simulink model "Geradeausfahrt"  (R2026b)
settings: Solver=FixedStepDiscrete  StopTime=inf  FixedStep=PAR_Sys_AbtastBasis_f64  EnableMultiTasking=on
StopFcn:
  | SpeichereGeradeausfahrt('Geradeausfahrt');
model workspace (MAT data in the model file):
  PAR_AktMot_PWM0_u8 = 80
  PAR_AktMot_RichtL_u8 = 0
  PAR_AktMot_RichtR_u8 = 1
  PAR_AktMot_Start_f32 = Simulink.Parameter
  PAR_AktMot_Start_f32.Value = 0
  PAR_AktMot_Start_f32.Complexity = 'real'
  PAR_AktMot_Start_f32.Dimensions = [1 1]
  PAR_AktMot_Start_f32.DataType = 'single'
  PAR_RegGer_Kp_f32 = Simulink.Parameter
  PAR_RegGer_Kp_f32.Value = 100
  PAR_RegGer_Kp_f32.Complexity = 'real'
  PAR_RegGer_Kp_f32.Dimensions = [1 1]
  PAR_RegGer_Kp_f32.DataType = 'single'
  PAR_RegGer_SSoll_f32 = 8
  PAR_SenOdo_IncU_f32 = 40
  PAR_SenOdo_KorrSL_f32 = 1
  PAR_SenOdo_RadR_f32 = 0.0320000015199
  PAR_SenOdo_Spur_f32 = 0.140000000596
  PAR_Sys_AbtastBasis_f64 = 0.01
  PAR_Sys_Abtast_f64 = 0.01
libraries: arduinolib x8
settings Model: SILPILModeSetting=veronly  SimulationMode=external
settings SolverCC: AutoInsertRateTranBlk=on
settings DataIOCC: ReturnWorkspaceOutputs=off
settings OptimizationCC: DifferentSizesBufferReuse=on  EfficientTunableParamExpr=on  EnhancedBackFolding=on  MaxStackSize=64  OptimizationCustomize=off  OptimizeBlockOrder=speed  PassReuseOutputArgsAs=Individual arguments  RemoveInternalMemoryZeroInit=on  RemoveRootLevelIOMemoryZeroInit=on
settings DebuggingCC: ParameterTunabilityLossMsg=error
settings HardwareCC: ProdHWDeviceType=ARM Compatible->ARM Cortex  ProdLargestAtomicFloat=Double  ProdLargestAtomicInteger=Long
settings SFSimCC: MATLABDynamicMemAlloc=off
settings RTWCC: BuildConfiguration=Faster Runs  Description=Embedded Coder  HardwareBoard=Arduino Uno R4 WiFi  SystemTargetFile=ert.tlc  TLCOptions=-aInlineSetEventsForThisBaseRateFcn=TLC_FALSE -aSuppressMultiTaskScheduler=TLC_FALSE -aRateBasedStepFcn=1  TemplateMakefile=ert_default_tmf  Toolchain=Arduino ARM M4
settings CodeAppCC: ForceParamTrailComments=on  IgnoreCustomStorageClasses=off  InsertBlockDesc=on  OperatorAnnotations=on  SFDataObjDesc=on  SimulinkDataObjDesc=on
settings ERTTargetCC: CombineSignalStateStructs=on  ExtModeAutomaticAllocSize=off  ExtModeIntrfLevel=Level2 - Open  ExtModeMexFile=ext_xcp  ExtModeStaticAlloc=on  SupportContinuousTime=on  SupportVariableSizeSignals=on

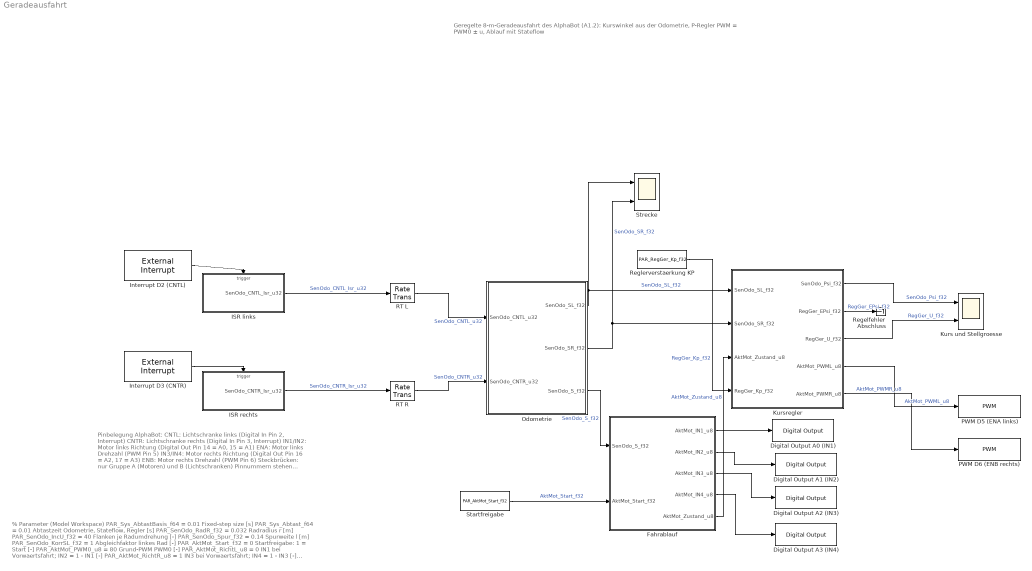
== system Geradeausfahrt ==
  note: % Parameter (Model Workspace)
      | PAR_Sys_AbtastBasis_f64 = 0.01 Fixed-step size [s]
      | PAR_Sys_Abtast_f64 = 0.01 Abtastzeit Odometrie, Stateflow, Regler [s]
      | PAR_SenOdo_RadR_f32 = 0.032 Radradius r [m]
      | PAR_SenOdo_IncU_f32 = 40 Flanken je Radumdrehung [-]
      | PAR_SenOdo_Spur_f32 = 0.14 Spurweite l [m]
      | PAR_SenOdo_KorrSL_f32 = 1 Abgleichfaktor linkes Rad [-]
      | PAR_AktMot_Start_f32 = 0 Startfreigabe: 1 = Start [-]
      | PAR_AktMot_PWM0_u8 = 80 Grund-PWM PWM0 [-]
      | PAR_AktMot_RichtL_u8 = 0 IN1 bei Vorwaertsfahrt; IN2 = 1 - IN1 [-]
      | PAR_AktMot_RichtR_u8 = 1 IN3 bei Vorwaertsfahrt; IN4 = 1 - IN3 [-]
      | PAR_RegGer_SSoll_f32 = 8 Sollstrecke [m]
      | PAR_RegGer_Kp_f32 = 100 Reglerverstae rkung KP [PWM/rad]
      |
      | % BSE_3: psi_k = psi_k-1 + (dsR - dsL) / l, e = 0 - psi, u = KP * e
      | PWML = PWM0 - u, PWMR = PWM0 + u
  note: Geregelte 8-m-Geradeausfahrt des AlphaBot (A1.2): Kurswinkel aus der Odometrie, P-Regler PWM = PWM0 ± u, Ablauf mit Stateflow
  note: Pinbelegung AlphaBot:
      | CNTL: Lichtschranke links (Digital In Pin 2, Interrupt)
      | CNTR: Lichtschranke rechts (Digital In Pin 3, Interrupt)
      | IN1/IN2: Motor links Richtung (Digital Out Pin 14 = A0, 15 = A1)
      | ENA: Motor links Drehzahl (PWM Pin 5)
      | IN3/IN4: Motor rechts Richtung (Digital Out Pin 16 = A2, 17 = A3)
      | ENB: Motor rechts Drehzahl (PWM Pin 6)
      | Steckbrücken: nur Gruppe A (Motoren) und B (Lichtschranken)
      | Pinnummern stehen direkt in den Blöcken (keine PAR_-Parameter).
  Digital Output A0 (IN1) : arduinolib/Digital Output  pinNumber=14  Direction=output  blockPlatform=arduino
  Digital Output A1 (IN2) : arduinolib/Digital Output  pinNumber=15  Direction=output  blockPlatform=arduino
  Digital Output A2 (IN3) : arduinolib/Digital Output  pinNumber=16  Direction=output  blockPlatform=arduino
  Digital Output A3 (IN4) : arduinolib/Digital Output  pinNumber=17  Direction=output  blockPlatform=arduino
  Fahrablauf : Stateflow chart  TreatAsAtomicUnit=on
  ISR links : Subsystem  TreatAsAtomicUnit=on
  ISR rechts : Subsystem  TreatAsAtomicUnit=on
  Interrupt D2 (CNTL) : arduinolib/External Interrupt  Pin=2  PullUp=off  Mode=CHANGE  InterruptSimulationInput=off
  Interrupt D3 (CNTR) : arduinolib/External Interrupt  Pin=3  PullUp=off  Mode=CHANGE  InterruptSimulationInput=off
  Kurs und Stellgroesse : Scope  NumInputPorts=2
      settings: ActiveDisplayYMinimum=-1.0587400176678445  ActiveDisplayYMaximum=1.3722724823321559
  Kursregler : MATLAB Function  TreatAsAtomicUnit=on
  Odometrie : MATLAB Function  TreatAsAtomicUnit=on
  PWM D5 (ENA links) : arduinolib/PWM  pinNumber=5  frequencyType=Default  desiredFrequency=490.2  achievableFrequency=490.2
  PWM D6 (ENB rechts) : arduinolib/PWM  pinNumber=6  frequencyType=Default  desiredFrequency=490.2  achievableFrequency=490.2
  RT L : RateTransition  Deterministic=off  OutPortSampleTime=PAR_Sys_Abtast_f64
  RT R : RateTransition  Deterministic=off  OutPortSampleTime=PAR_Sys_Abtast_f64
  Regelfehler Abschluss : Terminator
  Reglerverstaerkung KP : Constant  Value=PAR_RegGer_Kp_f32  OutDataTypeStr=single  SampleTime=PAR_Sys_Abtast_f64
  Startfreigabe : Constant  Value=PAR_AktMot_Start_f32  OutDataTypeStr=single  SampleTime=PAR_Sys_Abtast_f64
  Strecke : Scope  NumInputPorts=2
      settings: ActiveDisplayYMinimum=-0.329834002092661  ActiveDisplayYMaximum=1.9353644368944749
  wires:
  Interrupt D2 (CNTL)/1 -> ISR links/Trigger
  ISR links/1(SenOdo_CNTL_Isr_u32) -> RT L/1  "SenOdo_CNTL_Isr_u32"
  Interrupt D3 (CNTR)/1 -> ISR rechts/Trigger
  ISR rechts/1(SenOdo_CNTR_Isr_u32) -> RT R/1  "SenOdo_CNTR_Isr_u32"
  RT L/1 -> Odometrie/1(SenOdo_CNTL_u32)  "SenOdo_CNTL_u32"
  RT R/1 -> Odometrie/2(SenOdo_CNTR_u32)  "SenOdo_CNTR_u32"
  Odometrie/3(SenOdo_S_f32) -> Fahrablauf/1(SenOdo_S_f32)  "SenOdo_S_f32"
  Startfreigabe/1 -> Fahrablauf/2(AktMot_Start_f32)  "AktMot_Start_f32"
  Odometrie/1(SenOdo_SL_f32) -> Kursregler/1(SenOdo_SL_f32), Strecke/1  "SenOdo_SL_f32"
  Odometrie/2(SenOdo_SR_f32) -> Kursregler/2(SenOdo_SR_f32), Strecke/2  "SenOdo_SR_f32"
  Fahrablauf/5(AktMot_Zustand_u8) -> Kursregler/3(AktMot_Zustand_u8)  "AktMot_Zustand_u8"
  Reglerverstaerkung KP/1 -> Kursregler/4(RegGer_Kp_f32)  "RegGer_Kp_f32"
  Kursregler/4(AktMot_PWML_u8) -> PWM D5 (ENA links)/1  "AktMot_PWML_u8"
  Kursregler/5(AktMot_PWMR_u8) -> PWM D6 (ENB rechts)/1  "AktMot_PWMR_u8"
  Fahrablauf/1(AktMot_IN1_u8) -> Digital Output A0 (IN1)/1
  Fahrablauf/2(AktMot_IN2_u8) -> Digital Output A1 (IN2)/1
  Fahrablauf/3(AktMot_IN3_u8) -> Digital Output A2 (IN3)/1
  Fahrablauf/4(AktMot_IN4_u8) -> Digital Output A3 (IN4)/1
  Kursregler/1(SenOdo_Psi_f32) -> Kurs und Stellgroesse/1  "SenOdo_Psi_f32"
  Kursregler/3(RegGer_U_f32) -> Kurs und Stellgroesse/2  "RegGer_U_f32"
  Kursregler/2(RegGer_EPsi_f32) -> Regelfehler Abschluss/1  "RegGer_EPsi_f32"

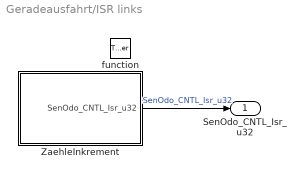
== system Geradeausfahrt/ISR links ==
  function : TriggerPort  TriggerType=function-call  VariantControl=(inherit)
  ZaehleInkrement : MATLAB Function  TreatAsAtomicUnit=on
  SenOdo_CNTL_Isr_u32 : Outport
  wires:
  ZaehleInkrement/1(SenOdo_CNTL_Isr_u32) -> SenOdo_CNTL_Isr_u32/1  "SenOdo_CNTL_Isr_u32"

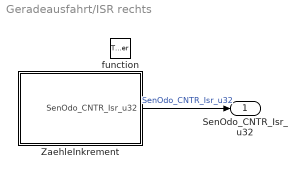
== system Geradeausfahrt/ISR rechts ==
  function : TriggerPort  TriggerType=function-call  VariantControl=(inherit)
  ZaehleInkrement : MATLAB Function  TreatAsAtomicUnit=on
  SenOdo_CNTR_Isr_u32 : Outport
  wires:
  ZaehleInkrement/1(SenOdo_CNTR_Isr_u32) -> SenOdo_CNTR_Isr_u32/1  "SenOdo_CNTR_Isr_u32"

== matlab function Geradeausfahrt/ISR rechts/ZaehleInkrement ==
  data: SenOdo_CNTR_Isr_u32 output
function SenOdo_CNTR_Isr_u32 = ZaehleInkrement()
% ZaehleInkrement: ISR je Flanke der Lichtschranke (Modus CHANGE)
% Ausgabe:  SenOdo_CNTR_Isr_u32 [1x1]: Flanken seit Programmstart [-]
persistent nZaehler   % Flankenzaehler [-]

if isempty(nZaehler)
    nZaehler = uint32(0);
end
nZaehler = nZaehler + 1;
SenOdo_CNTR_Isr_u32 = nZaehler;
end

== matlab function Geradeausfahrt/ISR links/ZaehleInkrement ==
  data: SenOdo_CNTL_Isr_u32 output
function SenOdo_CNTL_Isr_u32 = ZaehleInkrement()
% ZaehleInkrement: ISR je Flanke der Lichtschranke (Modus CHANGE)
% Ausgabe:  SenOdo_CNTL_Isr_u32 [1x1]: Flanken seit Programmstart [-]
persistent nZaehler   % Flankenzaehler [-]

if isempty(nZaehler)
    nZaehler = uint32(0);
end
nZaehler = nZaehler + 1;
SenOdo_CNTL_Isr_u32 = nZaehler;
end

== matlab function Geradeausfahrt/Odometrie ==
  settings: updateMethod=DISCRETE  sampleTime=PAR_Sys_Abtast_f64
  data: SenOdo_CNTL_u32 input; SenOdo_SL_f32 output; SenOdo_CNTR_u32 input; SenOdo_SR_f32 output; SenOdo_S_f32 output; PAR_SenOdo_RadR_f32 parameter; PAR_SenOdo_IncU_f32 parameter; PAR_SenOdo_KorrSL_f32 parameter
function [SenOdo_SL_f32,SenOdo_SR_f32,SenOdo_S_f32] = BerechneStrecke(SenOdo_CNTL_u32,SenOdo_CNTR_u32,PAR_SenOdo_RadR_f32,PAR_SenOdo_IncU_f32,PAR_SenOdo_KorrSL_f32)
% BerechneStrecke: Radstrecken und mittlere Strecke aus den Flankenzaehlern
% Eingabe:  SenOdo_CNTL_u32, SenOdo_CNTR_u32 [1x1]: Flanken links, rechts [-]
%           PAR_SenOdo_RadR_f32 Radradius [m], PAR_SenOdo_IncU_f32 Flanken je Umdrehung [-]
%           PAR_SenOdo_KorrSL_f32 Abgleichfaktor linkes Rad, Start 1 [-]
% Ausgabe:  SenOdo_SL_f32, SenOdo_SR_f32 [1x1]: Radstrecke links, rechts [m]
%           SenOdo_S_f32                 [1x1]: mittlere Strecke s = (sL + sR)/2 [m]
fWegInkrement = 2 * single(pi) * PAR_SenOdo_RadR_f32 / PAR_SenOdo_IncU_f32;   % Weg je Flanke [m]
SenOdo_SL_f32 = single(SenOdo_CNTL_u32) * fWegInkrement * PAR_SenOdo_KorrSL_f32;
SenOdo_SR_f32 = single(SenOdo_CNTR_u32) * fWegInkrement;
SenOdo_S_f32 = (SenOdo_SL_f32 + SenOdo_SR_f32) / 2;
end

== stateflow chart Geradeausfahrt/Fahrablauf ==
  settings: updateMethod=DISCRETE  sampleTime=PAR_Sys_Abtast_f64  executeAtInitialization=1
  state Stillstand
    entry:
    AktMot_IN1_u8 = uint8(0);
    AktMot_IN2_u8 = uint8(0);
    AktMot_IN3_u8 = uint8(0);
    AktMot_IN4_u8 = uint8(0);
    AktMot_Zustand_u8 = uint8(0);
  state Fahrt
    entry:
    AktMot_IN1_u8 = PAR_AktMot_RichtL_u8;
    AktMot_IN2_u8 = uint8(1) - PAR_AktMot_RichtL_u8;
    AktMot_IN3_u8 = PAR_AktMot_RichtR_u8;
    AktMot_IN4_u8 = uint8(1) - PAR_AktMot_RichtR_u8;
    AktMot_Zustand_u8 = uint8(1);
  state Stopp
    entry:
    AktMot_IN1_u8 = uint8(0);
    AktMot_IN2_u8 = uint8(0);
    AktMot_IN3_u8 = uint8(0);
    AktMot_IN4_u8 = uint8(0);
    AktMot_Zustand_u8 = uint8(2);
  (default) -> Stillstand
  Stillstand -> Fahrt : [AktMot_Start_f32 >= 1]
  Fahrt -> Stopp : [SenOdo_S_f32 >= PAR_RegGer_SSoll_f32]
  data: SenOdo_S_f32 input single; AktMot_Start_f32 input single; AktMot_IN1_u8 output uint8; AktMot_IN2_u8 output uint8; AktMot_IN3_u8 output uint8; AktMot_IN4_u8 output uint8; AktMot_Zustand_u8 output uint8; PAR_RegGer_SSoll_f32 parameter single; PAR_AktMot_RichtL_u8 parameter uint8; PAR_AktMot_RichtR_u8 parameter uint8

== matlab function Geradeausfahrt/Kursregler ==
  settings: updateMethod=DISCRETE  sampleTime=PAR_Sys_Abtast_f64
  data: SenOdo_SL_f32 input; SenOdo_Psi_f32 output; SenOdo_SR_f32 input; AktMot_Zustand_u8 input; RegGer_Kp_f32 input; RegGer_EPsi_f32 output; RegGer_U_f32 output; AktMot_PWML_u8 output; AktMot_PWMR_u8 output; PAR_SenOdo_Spur_f32 parameter; PAR_AktMot_PWM0_u8 parameter
function [SenOdo_Psi_f32,RegGer_EPsi_f32,RegGer_U_f32,AktMot_PWML_u8,AktMot_PWMR_u8] = RegleKurs(SenOdo_SL_f32,SenOdo_SR_f32,AktMot_Zustand_u8,RegGer_Kp_f32,PAR_SenOdo_Spur_f32, PAR_AktMot_PWM0_u8)
% RegleKurs: Kurswinkel aus der Odometrie und P-Regler auf den Sollkurs 0 rad
% Eingabe:  SenOdo_SL_f32, SenOdo_SR_f32 [1x1]: Radstrecke links, rechts [m]
%           AktMot_Zustand_u8 [1x1]: 0 Stillstand, 1 Fahrt, 2 Stopp [-]
%           RegGer_Kp_f32 [1x1]: Reglerverstaerkung KP [1/rad]
%           PAR_SenOdo_Spur_f32 Spurweite l [m], PAR_AktMot_PWM0_u8 Grund-PWM PWM0 [-]
% Ausgabe:  SenOdo_Psi_f32 [1x1]: Kurswinkel psi [rad], positiv nach links
%           RegGer_EPsi_f32 [1x1]: Regelfehler e = 0 - psi [rad]
%           RegGer_U_f32 [1x1]: Stellgroesse u = KP * e [-]
%           AktMot_PWML_u8, AktMot_PWMR_u8 [1x1]: PWM0 - u, PWM0 + u, begrenzt auf 0...255 [-]
persistent fPsi fSLAlt fSRAlt   % Kurswinkel [rad], Radstrecken im vorigen Schritt [m]

if isempty(fPsi)
    fPsi = single(0);
    fSLAlt = SenOdo_SL_f32;
    fSRAlt = SenOdo_SR_f32;
end
% psi_k = psi_k-1 + (dsR - dsL)/l; im Stillstand auf 0 gesetzt (Startrichtung = Sollkurs)
fDeltaPsi = ((SenOdo_SR_f32 - fSRAlt) - (SenOdo_SL_f32 - fSLAlt)) / PAR_SenOdo_Spur_f32;   % Kursaenderung [rad]
fSLAlt = SenOdo_SL_f32;
fSRAlt = SenOdo_SR_f32;
if AktMot_Zustand_u8 == 0
    fPsi = single(0);
else
    fPsi = fPsi + fDeltaPsi;
end
SenOdo_Psi_f32 = fPsi;
RegGer_EPsi_f32 = single(0) - fPsi;
RegGer_U_f32 = RegGer_Kp_f32 * RegGer_EPsi_f32;
% PWM = PWM0 -/+ u nur in Fahrt; uint8() rundet und begrenzt auf 0...255
AktMot_PWML_u8 = uint8(0);
AktMot_PWMR_u8 = uint8(0);
if AktMot_Zustand_u8 == 1
    AktMot_PWML_u8 = uint8(single(PAR_AktMot_PWM0_u8) - RegGer_U_f32);
    AktMot_PWMR_u8 = uint8(single(PAR_AktMot_PWM0_u8) + RegGer_U_f32);
end
end
